simulink model "model"  (R2025b)
settings: Solver=ode15s  StartTime=0.0  StopTime=10  MaxStep=1e-4  RelTol=1e-4
values from neighbouring files (symbols this model uses):
  A = [3 -1; -2 2]    [init.m]
  A_0g = [0     1 ... (first row only)    [init.m]
  B = [8; 8]    [init.m]
  B_0g = [0; 1]    [init.m]
  C = [1 0]    [init.m]
  gamma = 500    [init.m]
  K = [171.613219295 -159.128557999]    [init.m]
  x_0 = [1; 0]    [init.m]
  xi_g0 = [0; 0]    [init.m]
undefined symbols (not defined in the file or in its folder): den, num
settings Model: Creator=eva  LastModifiedBy=eva

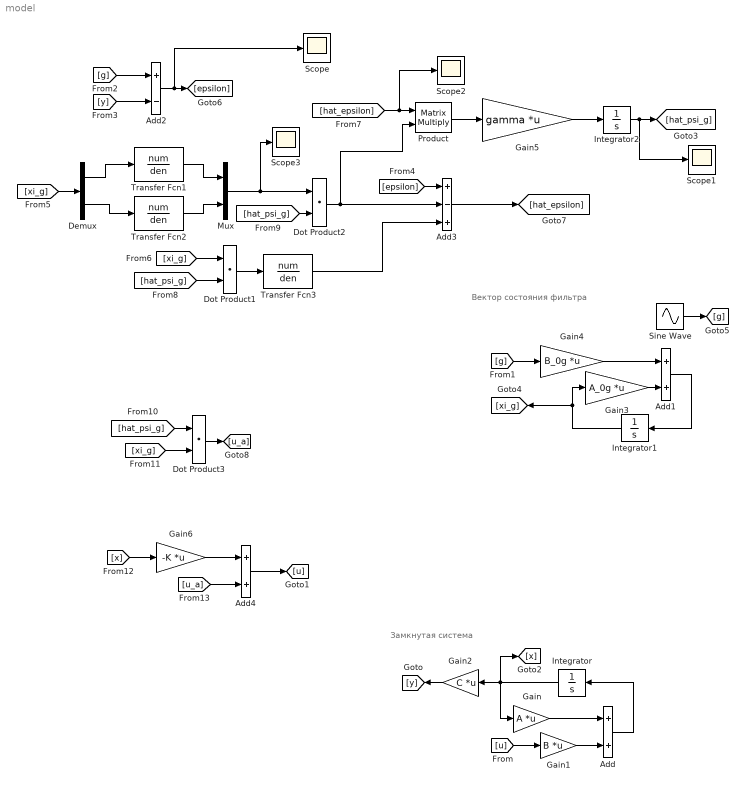
== system model ==
  note: Вектор состояния фильтра
  note: Замкнутая система
  Add : Sum
  Add1 : Sum
  Add2 : Sum  Inputs=+-
  Add3 : Sum  Inputs=+-+
  Add4 : Sum
  Demux : Demux  Outputs=2
  Dot Product1 : DotProduct  OutDataTypeStr=Inherit: Inherit via internal rule
  Dot Product2 : DotProduct  OutDataTypeStr=Inherit: Inherit via internal rule
  Dot Product3 : DotProduct  OutDataTypeStr=Inherit: Inherit via internal rule
  Gain : Gain  Gain=A  Multiplication=Matrix(K*u)
  Gain1 : Gain  Gain=B  Multiplication=Matrix(K*u)
  Gain2 : Gain  Gain=C  Multiplication=Matrix(K*u)
  Gain3 : Gain  Gain=A_0g  Multiplication=Matrix(K*u)
  Gain4 : Gain  Gain=B_0g  Multiplication=Matrix(K*u)
  Gain5 : Gain  Gain=gamma  Multiplication=Matrix(K*u)
  Gain6 : Gain  Gain=-K  Multiplication=Matrix(K*u)
  Integrator : Integrator  InitialCondition=x_0
  Integrator1 : Integrator  InitialCondition=xi_g0
  Integrator2 : Integrator  InitialCondition=xi_g0
  Mux : Mux  Inputs=2
  Product : Product  Multiplication=Matrix(*)
  Scope{,1..3} (4 alike) : Scope
      Scope settings: ActiveDisplayYMinimum=-1  ActiveDisplayYMaximum=1
      Scope1 settings: ActiveDisplayYMinimum=-0.068210261872114472  ActiveDisplayYMaximum=0.10261494344603757
      Scope2 settings: ActiveDisplayYMinimum=-6.2194720262212444  ActiveDisplayYMaximum=14.621196712926473  DataLoggingVariableName=ScopeData2
      Scope3 settings: ActiveDisplayYMinimum=-1.0733130483373419  ActiveDisplayYMaximum=2.4990957196297816  DataLoggingVariableName=ScopeData3
  Sine Wave : Sin  Amplitude=10  Bias=pi/2  Frequency=8  Phase=1  SampleTime=0
  Transfer Fcn1 : TransferFcn  Numerator=num  Denominator=den
  Transfer Fcn2 : TransferFcn  Numerator=num  Denominator=den
  Transfer Fcn3 : TransferFcn  Numerator=num  Denominator=den
  wires:
  [u] -> Gain1/1
  Gain1/1 -> Add/2
  Gain/1 -> Add/1
  Add/1 -> Integrator/1
  Gain2/1 -> [y]
  Gain4/1 -> Add1/1
  Gain3/1 -> Add1/2
  Add1/1 -> Integrator1/1
  Integrator1/1 -> [xi_g], Gain3/1
  Sine Wave/1 -> [g]
  [g] -> Gain4/1
  [g] -> Add2/1
  [y] -> Add2/2
  Add2/1 -> Scope/1, [epsilon]
  [xi_g] -> Demux/1
  Demux/1 -> Transfer Fcn1/1
  Transfer Fcn2/1 -> Mux/2
  Transfer Fcn1/1 -> Mux/1
  Dot Product2/1 -> Product/2, Add3/2
  [xi_g] -> Dot Product1/1
  [hat_psi_g] -> Dot Product1/2
  Dot Product1/1 -> Transfer Fcn3/1
  Transfer Fcn3/1 -> Add3/3
  [epsilon] -> Add3/1
  Add3/1 -> [hat_epsilon]
  [hat_epsilon] -> Scope2/1, Product/1
  Product/1 -> Gain5/1
  Gain5/1 -> Integrator2/1
  Mux/1 -> Scope3/1, Dot Product2/1
  [hat_psi_g] -> Dot Product2/2
  [hat_psi_g] -> Dot Product3/1
  [xi_g] -> Dot Product3/2
  Dot Product3/1 -> [u_a]
  Demux/2 -> Transfer Fcn2/1
  [x] -> Gain6/1
  Gain6/1 -> Add4/1
  [u_a] -> Add4/2
  Add4/1 -> [u]
  Integrator/1 -> Gain2/1, [x], Gain/1
  Integrator2/1 -> Scope1/1, [hat_psi_g]
